simulink model "Akilli_Sayac"  (R2026b)
settings: Solver=ode23t  StopTime=t_stop  MaxStep=1e-4  RelTol=1e-4
InitFcn:
  | akilli_sayac_param
values from neighbouring files (symbols this model uses):
  bulasik_t = [0   22.5   25]    [akilli_sayac_param.m]
  bulasik_u = [0   1      0 ]    [akilli_sayac_param.m]
  camasir_t = [0   19   20.5   25]    [akilli_sayac_param.m]
  camasir_u = [0   1    0      0 ]    [akilli_sayac_param.m]
  firin_t = [0   18   19   25]    [akilli_sayac_param.m]
  firin_u = [0   1    0    0 ]    [akilli_sayac_param.m]
  k_kWh = 3600/3.6e6    (= 0.001)    [akilli_sayac_param.m]
  kap_t = [0 25]    [akilli_sayac_param.m]
  kap_u = [0 0]    [akilli_sayac_param.m]
  kettle_t = [0   7   7+10*dk   18   18+10*dk   25]    [akilli_sayac_param.m]
  kettle_u = [0   1   0         1    0          0 ]    [akilli_sayac_param.m]
  klima_t = [0   20   23   25]    [akilli_sayac_param.m]
  klima_u = [0   1    0    0 ]    [akilli_sayac_param.m]
  R_baz = Vrms^2*pf_baz^2/P_baz    (= 225.706666667)    [akilli_sayac_param.m]
  R_bulasik = Vrms^2/P_bulasik    (= 40.0757575758)    [akilli_sayac_param.m]
  R_camasir = Vrms^2*pf_camasir^2/P_camasir    (= 24.1828571429)    [akilli_sayac_param.m]
  R_firin = Vrms^2/P_firin    (= 22.0416666667)    [akilli_sayac_param.m]
  R_kettle = Vrms^2/P_kettle    (= 26.45)    [akilli_sayac_param.m]
  R_klima = Vrms^2*pf_klima^2/P_klima    (= 33.5265350877)    [akilli_sayac_param.m]
  R_tv = Vrms^2/P_tv    (= 637.34939759)    [akilli_sayac_param.m]
  T1_t = [0  6 17 25]    [akilli_sayac_param.m]
  T1_u = [0 1 0 0]    [akilli_sayac_param.m]
  T2_t = [0 17 22 25]    [akilli_sayac_param.m]
  T2_u = [0 1 0 0]    [akilli_sayac_param.m]
  T3_t = [0  6 22 25]    [akilli_sayac_param.m]
  T3_u = [1 0 1 1]    [akilli_sayac_param.m]
  t_kesme = 25    [akilli_sayac_param.m]
  tv_t = [0   19   25]    [akilli_sayac_param.m]
  tv_u = [0   1    0 ]    [akilli_sayac_param.m]
libraries: fl_lib x23, nesl_utility x11, eeRmsMeasurement x2, eePowerMeasurement x1
settings Model: Creator=Poyraz  LastModifiedBy=Poyraz
settings SimscapeCC: SimscapeLogType=all  SimscapeNominalValues="[{\"value\":\"1\",\"unit\":\"A\"},{\"value\":\"1\",\"unit\":\"bar\"},{\"value\":\"1\",\"unit\":\"cm^2\"},{\"value\":\"1\",\"unit\":\"cm^3/s\"},{\"value\":\"1\",\"unit\":\"kJ/kg\"},{\"value\":\"1\",\"unit\":\"kW\"},{\"value\":\"1\",\"unit\":\"l\"},{\"value\":\"1\",\"unit\":\"N\"},{\"value\":\"1\",\"unit\":\"N*m\"},{\"value\":\"1\",\"unit\":\"V\"},{\"value\":\"0.001\",\"unit\":\"Wb\"}]"  SimscapeUseEnergyAccounting=off

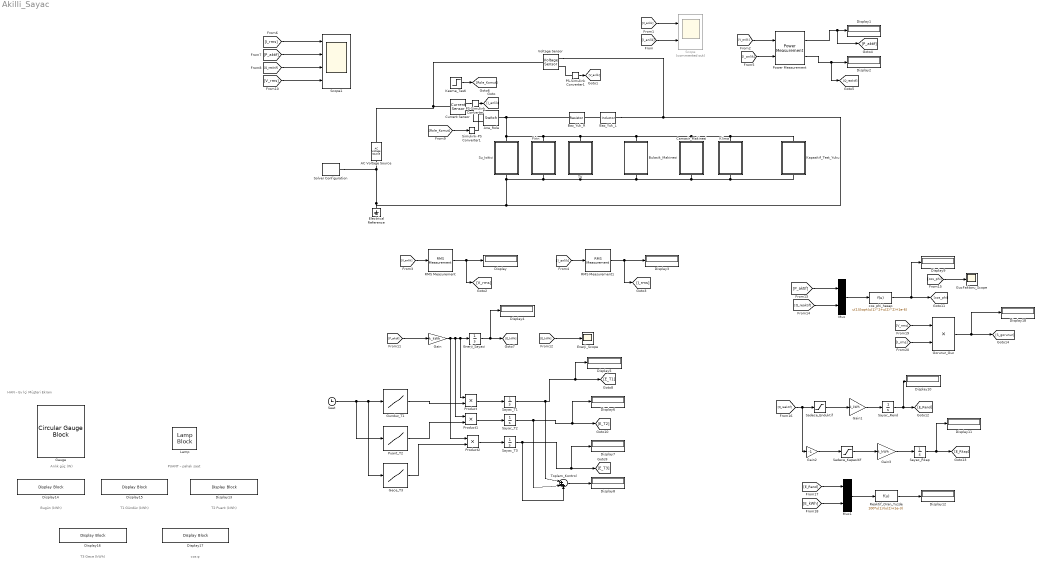
== system Akilli_Sayac ==
  note: cos φ
  note: T3 Gece (kWh)
  note: T2 Puant (kWh)
  note: T1 Gündüz (kWh)
  note: Bugün (kWh)
  note: PUANT – pahalı saat
  note: Anlık güç (W)
  note: HAN – Ev İçi Müşteri Ekranı
  AC Voltage Source : fl_lib/Electrical/Electrical Sources/AC Voltage Source  amp=Vpk V  shift=0 deg  frequency=f Hz
  Ana_Role : fl_lib/Electrical/Electrical Elements/Switch  R_closed=0.01 Ohm  G_open=1e-8 1/Ohm  Threshold=0.5  i_specify=off  i_priority=None  i=0 A  i_nominal_specify=off  i_nominal_value=1  i_nominal_unit=A  v_specify=off  v_priority=None  v=0 V  v_nominal_specify=off  v_nominal_value=1  v_nominal_unit=V
  Baz_Yuk_L : fl_lib/Electrical/Electrical Elements/Inductor  l=L_baz H  r=0 Ohm  g=1e-4 1/Ohm  i_specify=off  i_priority=None  i=0 A  i_nominal_specify=off  i_nominal_value=1  i_nominal_unit=A  v_specify=off  v_priority=None  v=0 V  v_nominal_specify=off  v_nominal_value=1  v_nominal_unit=V  i_L_specify=off  i_L_priority=High  i_L=0 A  i_L_nominal_specify=off  i_L_nominal_value=1  i_L_nominal_unit=A
  Baz_Yuk_R : fl_lib/Electrical/Electrical Elements/Resistor  R=R_baz Ohm  i_specify=off  i_priority=None  i=0 A  i_nominal_specify=off  i_nominal_value=1  i_nominal_unit=A  v_specify=off  v_priority=None  v=0 V  v_nominal_specify=off  v_nominal_value=1  v_nominal_unit=V
  Bulasik_Makinesi : Subsystem
  Camasir_Makinesi : Subsystem
  Current Sensor : fl_lib/Electrical/Electrical Sensors/Current Sensor
  Display{,1..12,18} (14 alike) : Display
  Display{13..17} (5 alike) : DisplayBlock  LabelPosition=Hide  Transparency=1  GridColor=[0.502, 0.502, 0.502]
  Electrical Reference : fl_lib/Electrical/Electrical Elements/Electrical Reference
  Enerji_Sayaci : Integrator
  Enerji_Scope : Scope
      settings: SampleTime=5e-3  ActiveDisplayYMinimum=-3.0259630448584041  ActiveDisplayYMaximum=17.0297155830163  DataLoggingVariableName=ScopeData2
  Firin : Subsystem
  Gain : Gain  Gain=k_kWh
  Gain1 : Gain  Gain=k_kWh
  Gain2 : Gain  Gain=-1
  Gain3 : Gain  Gain=k_kWh
  Gauge : CircularGaugeBlock  ScaleMax=5000  TickInterval=500  FontColor=[0.0, 0.0, 0.0]
  Gece_T3 : Lookup_n-D  NumberOfTableDimensions=1  BreakpointsForDimension1=T3_t  Table=T3_u  InterpMethod=Flat  InternalRulePriority=Speed  RndMeth=Simplest
  Gorunur_Guc : Product
  GucFaktoru_Scope : Scope
      settings: SampleTime=5e-3  ActiveDisplayYMinimum=-0.16470130830471796  ActiveDisplayYMaximum=1.1474107836524428  DataLoggingVariableName=ScopeData3
  Gunduz_T1 : Lookup_n-D  NumberOfTableDimensions=1  BreakpointsForDimension1=T1_t  Table=T1_u  InterpMethod=Flat  InternalRulePriority=Speed  RndMeth=Simplest
  Kapasitif_Test_Yuku : Subsystem
  Kesme_Testi : Step  Time=t_kesme  InitialValue=1  FinalValue=0  SampleTime=0
  Klima : Subsystem
  Lamp : LampBlock  LabelPosition=Hide  DefaultColor=[192.0, 192.0, 192.0]
  Mux : Mux  Inputs=2
  Mux1 : Mux  Inputs=2
  PS-Simulink Converter : nesl_utility/PS-Simulink Converter  PhysicalDomain=network_engine_domain  SubClassName=ps_output  LeftPortType=input  RightPortType=output  PseudoPeriodic=off  Frequencies=[]  VectorFormat=inherit  Unit=A  AffineConversion=off
  PS-Simulink Converter1 : nesl_utility/PS-Simulink Converter  PhysicalDomain=network_engine_domain  SubClassName=ps_output  LeftPortType=input  RightPortType=output  PseudoPeriodic=off  Frequencies=[]  VectorFormat=inherit  Unit=V  AffineConversion=off
  Power Measurement : eePowerMeasurement/Power Measurement  LabelModeActiveChoice=Continuous  F=f  K=[1]  Ts=0
  Product : Product
  Product1 : Product
  Product2 : Product
  Puant_T2 : Lookup_n-D  NumberOfTableDimensions=1  BreakpointsForDimension1=T2_t  Table=T2_u  InterpMethod=Flat  InternalRulePriority=Speed  RndMeth=Simplest
  RMS Measurement : eeRmsMeasurement/RMS Measurement  LabelModeActiveChoice=Total  F=f  SpecifyHarmonics=off  K=[0 1 2]  InitialRMS=0  Ts=0
      settings: LibrarySourceBlock=|
      | ee_sl_lib/Measurements/RMS
      | Measurement
  RMS Measurement1 : eeRmsMeasurement/RMS Measurement  LabelModeActiveChoice=Total  F=f  SpecifyHarmonics=off  K=[0 1 2]  InitialRMS=0  Ts=0
      settings: LibrarySourceBlock=|
      | ee_sl_lib/Measurements/RMS
      | Measurement
  Reaktif_Oran_Yuzde : Fcn  Expr=100*u(1)/(u(2)+1e-3)
  Saat : Clock
  Sadece_Enduktif : Saturate  UpperLimit=inf  LowerLimit=0
  Sadece_Kapasitif : Saturate  UpperLimit=Inf  LowerLimit=0
  Sayac_Rend : Integrator
  Sayac_Rkap : Integrator
  Sayac_T1 : Integrator
  Sayac_T2 : Integrator
  Sayac_T3 : Integrator
  Scope : Scope  Commented=on  NumInputPorts=2
      settings: ActiveDisplayYMinimum=-398.438375066242  ActiveDisplayYMaximum=373.58690131662831
  Scope1 : Scope  NumInputPorts=4
      settings: SampleTime=5e-3  ActiveDisplayYMinimum=0.41959771500038417  ActiveDisplayYMaximum=4.3103626039758209
  Simulink-PS Converter1 : nesl_utility/Simulink-PS Converter  PhysicalDomain=network_engine_domain  SubClassName=ps_input  LeftPortType=input  RightPortType=output  PseudoPeriodic=off  Frequencies=[]  NoiseDistribution=none  NoiseParameters=[]  Unit=1  AffineConversion=off  FilteringAndDerivatives=provide  SimscapeFilterOrder=1  InputFilterTimeConstant=0.001  UdotUserProvided=0
  Solver Configuration : nesl_utility/Solver Configuration  PhysicalDomain=network_engine_domain  SubClassName=solver  LeftPortType=input  RightPortType=generic  Tones=[]  Harmonics=[]  SimulateNoise=off  Profile=off  UseLocalSampling=off  EnableSwitchedLinearOptims=on  FrequencyDomain=off  UseCCode=off  RelTol=0.001  AbsTol=0.001  MinStep=1e-09  ToWorkspace=off  RevertToSquareIcSolve=off  NumHomotopyIterations=100  PhasorMode=off  PhasorModeNumHarmonics=1  ConsistencySolver=NEWTON_XTOL_AFTER_FTOL  CanonicalOrdering=CANONICAL  OptimizeIntermediates=OPTIMIZED  MulticoreSolverChoice=BACKWARD_EULER  IndexReductionMethod=DerivativeReplacement  DoDC=off  ResidualTolerance=1e-09  ConsistencyTolSource=GLOBAL  ConsistencyAbsTol=0.001  ConsistencyRelTol=0.001  ConsistencyTolFactor=0.001  UseLocalSolver=off  LocalSolverChoice=NE_BACKWARD_EULER_ADVANCER  ResolveIndetEquations=on  FunctionEvalNumThread=1  LocalSolverSampleTime=0.001  DoFixedCost=off  MaxNonlinIter=3  MaxModeIter=2  ComputeImpulses=off  ImpulseIterations=2  LinearAlgebra=auto  LinearAlgebraNumThread=0  EquationFormulation=NE_TIME_EF  DelaysMemoryBudget=1024  AutomaticFiltering=on  FilteringTimeConstant=0.001  PartitionStorageMethod=AS_NEEDED  PartitionMemoryBudget=1024  PartitionMethod=BALANCED  MultibodyUseLocalSolver=off  MultibodyLocalSolverChoice=ODE1  MultibodyLocalSolverSampleTime=0.001
  Su_Isitici : Subsystem
  TV : Subsystem
  Toplam_Kontrol : Sum  Inputs=|+++
  Voltage Sensor : fl_lib/Electrical/Electrical Sensors/Voltage Sensor
  cos_phi_hesap : Fcn  Expr=u(1)/(sqrt(u(1)^2+u(2)^2)+1e-6)
  wires:
  PS-Simulink Converter1/1 -> [V_anlik]
  PS-Simulink Converter/1 -> [I_anlik]
  [V_anlik] -> Scope/1
  [I_anlik] -> Scope/2
  [V_anlik] -> RMS Measurement/1
  [I_anlik] -> RMS Measurement1/1
  RMS Measurement/1 -> [V_rms], Display/1
  RMS Measurement1/1 -> [I_rms], Display3/1
  [I_anlik] -> Power Measurement/2
  Power Measurement/2 -> [Q_reaktif], Display2/1
  Power Measurement/1 -> [P_aktif], Display1/1
  [I_rms] -> Scope1/1
  [P_aktif] -> Scope1/2
  [Q_reaktif] -> Scope1/3
  Kesme_Testi/1 -> [Role_Komut]
  [Role_Komut] -> Simulink-PS Converter1/1
  [V_rms] -> Scope1/4
  [P_aktif] -> Gain/1
  Gain/1 -> Product2/1, Product1/1, Product/1, Enerji_Sayaci/1
  Enerji_Sayaci/1 -> Display4/1, [E_kWh]
  [E_kWh] -> Enerji_Scope/1
  [V_anlik] -> Power Measurement/1
  Saat/1 -> Puant_T2/1, Gece_T3/1, Gunduz_T1/1
  Gunduz_T1/1 -> Product/2
  Puant_T2/1 -> Product1/2
  Gece_T3/1 -> Product2/2
  Product2/1 -> Sayac_T3/1
  Product1/1 -> Sayac_T2/1
  Product/1 -> Sayac_T1/1
  Sayac_T1/1 -> Toplam_Kontrol/1, Display5/1, [E_T1]
  Sayac_T2/1 -> Toplam_Kontrol/2, Display6/1, [E_T2]
  Sayac_T3/1 -> Toplam_Kontrol/3, Display7/1, [E_T3]
  Toplam_Kontrol/1 -> Display8/1
  [P_aktif] -> Mux/1
  [Q_reaktif] -> Mux/2
  Mux/1 -> cos_phi_hesap/1
  cos_phi_hesap/1 -> Display9/1, [cos_phi]
  [cos_phi] -> GucFaktoru_Scope/1
  [Q_reaktif] -> Gain2/1, Sadece_Enduktif/1
  Sadece_Enduktif/1 -> Gain1/1
  Gain1/1 -> Sayac_Rend/1
  Sayac_Rend/1 -> Display10/1, [E_Rend]
  Gain2/1 -> Sadece_Kapasitif/1
  Sadece_Kapasitif/1 -> Gain3/1
  Gain3/1 -> Sayac_Rkap/1
  Sayac_Rkap/1 -> Display11/1, [E_Rkap]
  [E_Rend] -> Mux1/1
  [E_kWh] -> Mux1/2
  Mux1/1 -> Reaktif_Oran_Yuzde/1
  Reaktif_Oran_Yuzde/1 -> Display12/1
  [I_rms] -> Gorunur_Guc/2
  [V_rms] -> Gorunur_Guc/1
  Gorunur_Guc/1 -> Display18/1, [S_gorunur]
  connections:
  AC Voltage Source/LConn1 -- Voltage Sensor/LConn1 -- Current Sensor/LConn1
  Baz_Yuk_L/LConn1 -- Baz_Yuk_R/RConn1
  Current Sensor/RConn1 -- PS-Simulink Converter/LConn1
  PS-Simulink Converter1/LConn1 -- Voltage Sensor/RConn1
  Current Sensor/RConn2 -- Ana_Role/RConn2
  Ana_Role/LConn1 -- Kapasitif_Test_Yuku/LConn1 -- Klima/LConn1 -- Camasir_Makinesi/LConn1 -- Bulasik_Makinesi/LConn1 -- TV/LConn1 -- Firin/LConn1 -- Su_Isitici/LConn1 -- Baz_Yuk_R/LConn1
  Ana_Role/RConn1 -- Simulink-PS Converter1/RConn1
  Electrical Reference/LConn1 -- Kapasitif_Test_Yuku/RConn1 -- Klima/RConn1 -- Camasir_Makinesi/RConn1 -- Bulasik_Makinesi/RConn1 -- TV/RConn1 -- Firin/RConn1 -- Su_Isitici/RConn1 -- Baz_Yuk_L/RConn1 -- Voltage Sensor/RConn2 -- Solver Configuration/RConn1 -- AC Voltage Source/RConn1

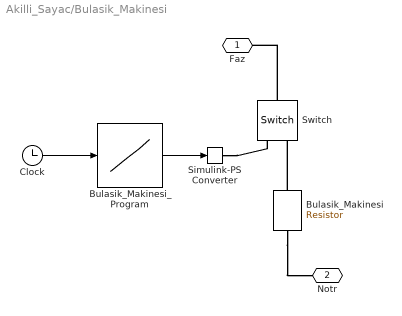
== system Akilli_Sayac/Bulasik_Makinesi ==
  Bulasik_Makinesi : fl_lib/Electrical/Electrical Elements/Resistor  R=R_bulasik Ohm  i_specify=off  i_priority=None  i=0 A  i_nominal_specify=off  i_nominal_value=1  i_nominal_unit=A  v_specify=off  v_priority=None  v=0 V  v_nominal_specify=off  v_nominal_value=1  v_nominal_unit=V
  Bulasik_Makinesi_Program : Lookup_n-D  NumberOfTableDimensions=1  BreakpointsForDimension1=bulasik_t  Table=bulasik_u  InterpMethod=Flat  InternalRulePriority=Speed  RndMeth=Simplest
  Clock : Clock
  Simulink-PS Converter : nesl_utility/Simulink-PS Converter  PhysicalDomain=network_engine_domain  SubClassName=ps_input  LeftPortType=input  RightPortType=output  PseudoPeriodic=off  Frequencies=[]  NoiseDistribution=none  NoiseParameters=[]  Unit=1  AffineConversion=off  FilteringAndDerivatives=provide  SimscapeFilterOrder=1  InputFilterTimeConstant=0.001  UdotUserProvided=0
  Switch : fl_lib/Electrical/Electrical Elements/Switch  R_closed=0.01 Ohm  G_open=1e-8 1/Ohm  Threshold=0.5  i_specify=off  i_priority=None  i=0 A  i_nominal_specify=off  i_nominal_value=1  i_nominal_unit=A  v_specify=off  v_priority=None  v=0 V  v_nominal_specify=off  v_nominal_value=1  v_nominal_unit=V
  Faz : PMIOPort  Side=Left
  Notr : PMIOPort  Port=2  Side=Right
  wires:
  Clock/1 -> Bulasik_Makinesi_Program/1
  Bulasik_Makinesi_Program/1 -> Simulink-PS Converter/1
  connections:
  Bulasik_Makinesi/RConn1 -- Notr/RConn1
  Bulasik_Makinesi/LConn1 -- Switch/RConn2
  Switch/LConn1 -- Faz/RConn1
  Simulink-PS Converter/RConn1 -- Switch/RConn1

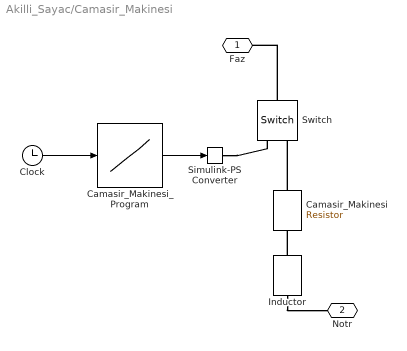
== system Akilli_Sayac/Camasir_Makinesi ==
  Camasir_Makinesi : fl_lib/Electrical/Electrical Elements/Resistor  R=R_camasir Ohm  i_specify=off  i_priority=None  i=0 A  i_nominal_specify=off  i_nominal_value=1  i_nominal_unit=A  v_specify=off  v_priority=None  v=0 V  v_nominal_specify=off  v_nominal_value=1  v_nominal_unit=V
  Camasir_Makinesi_Program : Lookup_n-D  NumberOfTableDimensions=1  BreakpointsForDimension1=camasir_t  Table=camasir_u  InterpMethod=Flat  InternalRulePriority=Speed  RndMeth=Simplest
  Clock : Clock
  Inductor : fl_lib/Electrical/Electrical Elements/Inductor  l=L_camasir H  r=0 Ohm  g=1e-4 1/Ohm  i_specify=off  i_priority=None  i=0 A  i_nominal_specify=off  i_nominal_value=1  i_nominal_unit=A  v_specify=off  v_priority=None  v=0 V  v_nominal_specify=off  v_nominal_value=1  v_nominal_unit=V  i_L_specify=off  i_L_priority=High  i_L=0 A  i_L_nominal_specify=off  i_L_nominal_value=1  i_L_nominal_unit=A
  Simulink-PS Converter : nesl_utility/Simulink-PS Converter  PhysicalDomain=network_engine_domain  SubClassName=ps_input  LeftPortType=input  RightPortType=output  PseudoPeriodic=off  Frequencies=[]  NoiseDistribution=none  NoiseParameters=[]  Unit=1  AffineConversion=off  FilteringAndDerivatives=provide  SimscapeFilterOrder=1  InputFilterTimeConstant=0.001  UdotUserProvided=0
  Switch : fl_lib/Electrical/Electrical Elements/Switch  R_closed=0.01 Ohm  G_open=1e-8 1/Ohm  Threshold=0.5  i_specify=off  i_priority=None  i=0 A  i_nominal_specify=off  i_nominal_value=1  i_nominal_unit=A  v_specify=off  v_priority=None  v=0 V  v_nominal_specify=off  v_nominal_value=1  v_nominal_unit=V
  Faz : PMIOPort  Side=Left
  Notr : PMIOPort  Port=2  Side=Right
  wires:
  Clock/1 -> Camasir_Makinesi_Program/1
  Camasir_Makinesi_Program/1 -> Simulink-PS Converter/1
  connections:
  Camasir_Makinesi/LConn1 -- Switch/RConn2
  Switch/LConn1 -- Faz/RConn1
  Simulink-PS Converter/RConn1 -- Switch/RConn1
  Inductor/LConn1 -- Camasir_Makinesi/RConn1
  Inductor/RConn1 -- Notr/RConn1

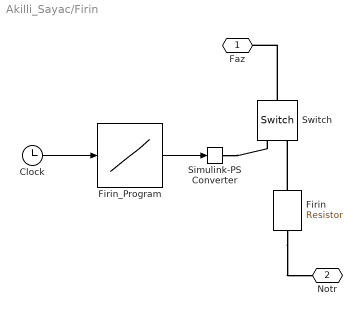
== system Akilli_Sayac/Firin ==
  Clock : Clock
  Firin : fl_lib/Electrical/Electrical Elements/Resistor  R=R_firin Ohm  i_specify=off  i_priority=None  i=0 A  i_nominal_specify=off  i_nominal_value=1  i_nominal_unit=A  v_specify=off  v_priority=None  v=0 V  v_nominal_specify=off  v_nominal_value=1  v_nominal_unit=V
  Firin_Program : Lookup_n-D  NumberOfTableDimensions=1  BreakpointsForDimension1=firin_t  Table=firin_u  InterpMethod=Flat  InternalRulePriority=Speed  RndMeth=Simplest
  Simulink-PS Converter : nesl_utility/Simulink-PS Converter  PhysicalDomain=network_engine_domain  SubClassName=ps_input  LeftPortType=input  RightPortType=output  PseudoPeriodic=off  Frequencies=[]  NoiseDistribution=none  NoiseParameters=[]  Unit=1  AffineConversion=off  FilteringAndDerivatives=provide  SimscapeFilterOrder=1  InputFilterTimeConstant=0.001  UdotUserProvided=0
  Switch : fl_lib/Electrical/Electrical Elements/Switch  R_closed=0.01 Ohm  G_open=1e-8 1/Ohm  Threshold=0.5  i_specify=off  i_priority=None  i=0 A  i_nominal_specify=off  i_nominal_value=1  i_nominal_unit=A  v_specify=off  v_priority=None  v=0 V  v_nominal_specify=off  v_nominal_value=1  v_nominal_unit=V
  Faz : PMIOPort  Side=Left
  Notr : PMIOPort  Port=2  Side=Right
  wires:
  Clock/1 -> Firin_Program/1
  Firin_Program/1 -> Simulink-PS Converter/1
  connections:
  Firin/RConn1 -- Notr/RConn1
  Firin/LConn1 -- Switch/RConn2
  Switch/LConn1 -- Faz/RConn1
  Simulink-PS Converter/RConn1 -- Switch/RConn1

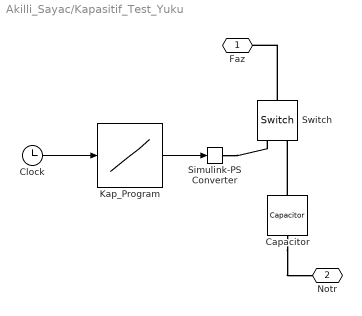
== system Akilli_Sayac/Kapasitif_Test_Yuku ==
  Capacitor : fl_lib/Electrical/Electrical Elements/Capacitor  c=C_kap F  r=1e-6 Ohm  g=0 1/Ohm  i_specify=off  i_priority=None  i=0 A  i_nominal_specify=off  i_nominal_value=1  i_nominal_unit=A  v_specify=off  v_priority=None  v=0 V  v_nominal_specify=off  v_nominal_value=1  v_nominal_unit=V  vc_specify=off  vc_priority=High  vc=0 V  vc_nominal_specify=off  vc_nominal_value=1  vc_nominal_unit=V
  Clock : Clock
  Kap_Program : Lookup_n-D  NumberOfTableDimensions=1  BreakpointsForDimension1=kap_t  Table=kap_u  InterpMethod=Flat  InternalRulePriority=Speed  RndMeth=Simplest
  Simulink-PS Converter : nesl_utility/Simulink-PS Converter  PhysicalDomain=network_engine_domain  SubClassName=ps_input  LeftPortType=input  RightPortType=output  PseudoPeriodic=off  Frequencies=[]  NoiseDistribution=none  NoiseParameters=[]  Unit=1  AffineConversion=off  FilteringAndDerivatives=provide  SimscapeFilterOrder=1  InputFilterTimeConstant=0.001  UdotUserProvided=0
  Switch : fl_lib/Electrical/Electrical Elements/Switch  R_closed=0.01 Ohm  G_open=1e-8 1/Ohm  Threshold=0.5  i_specify=off  i_priority=None  i=0 A  i_nominal_specify=off  i_nominal_value=1  i_nominal_unit=A  v_specify=off  v_priority=None  v=0 V  v_nominal_specify=off  v_nominal_value=1  v_nominal_unit=V
  Faz : PMIOPort  Side=Left
  Notr : PMIOPort  Port=2  Side=Right
  wires:
  Clock/1 -> Kap_Program/1
  Kap_Program/1 -> Simulink-PS Converter/1
  connections:
  Switch/LConn1 -- Faz/RConn1
  Simulink-PS Converter/RConn1 -- Switch/RConn1
  Capacitor/LConn1 -- Switch/RConn2
  Capacitor/RConn1 -- Notr/RConn1

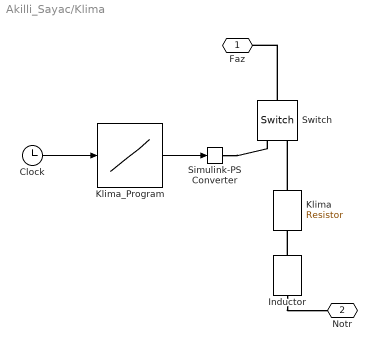
== system Akilli_Sayac/Klima ==
  Clock : Clock
  Inductor : fl_lib/Electrical/Electrical Elements/Inductor  l=L_klima H  r=0 Ohm  g=1e-4 1/Ohm  i_specify=off  i_priority=None  i=0 A  i_nominal_specify=off  i_nominal_value=1  i_nominal_unit=A  v_specify=off  v_priority=None  v=0 V  v_nominal_specify=off  v_nominal_value=1  v_nominal_unit=V  i_L_specify=off  i_L_priority=High  i_L=0 A  i_L_nominal_specify=off  i_L_nominal_value=1  i_L_nominal_unit=A
  Klima : fl_lib/Electrical/Electrical Elements/Resistor  R=R_klima Ohm  i_specify=off  i_priority=None  i=0 A  i_nominal_specify=off  i_nominal_value=1  i_nominal_unit=A  v_specify=off  v_priority=None  v=0 V  v_nominal_specify=off  v_nominal_value=1  v_nominal_unit=V
  Klima_Program : Lookup_n-D  NumberOfTableDimensions=1  BreakpointsForDimension1=klima_t  Table=klima_u  InterpMethod=Flat  InternalRulePriority=Speed  RndMeth=Simplest
  Simulink-PS Converter : nesl_utility/Simulink-PS Converter  PhysicalDomain=network_engine_domain  SubClassName=ps_input  LeftPortType=input  RightPortType=output  PseudoPeriodic=off  Frequencies=[]  NoiseDistribution=none  NoiseParameters=[]  Unit=1  AffineConversion=off  FilteringAndDerivatives=provide  SimscapeFilterOrder=1  InputFilterTimeConstant=0.001  UdotUserProvided=0
  Switch : fl_lib/Electrical/Electrical Elements/Switch  R_closed=0.01 Ohm  G_open=1e-8 1/Ohm  Threshold=0.5  i_specify=off  i_priority=None  i=0 A  i_nominal_specify=off  i_nominal_value=1  i_nominal_unit=A  v_specify=off  v_priority=None  v=0 V  v_nominal_specify=off  v_nominal_value=1  v_nominal_unit=V
  Faz : PMIOPort  Side=Left
  Notr : PMIOPort  Port=2  Side=Right
  wires:
  Clock/1 -> Klima_Program/1
  Klima_Program/1 -> Simulink-PS Converter/1
  connections:
  Klima/LConn1 -- Switch/RConn2
  Switch/LConn1 -- Faz/RConn1
  Simulink-PS Converter/RConn1 -- Switch/RConn1
  Inductor/LConn1 -- Klima/RConn1
  Inductor/RConn1 -- Notr/RConn1

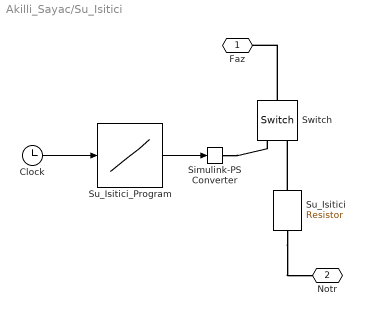
== system Akilli_Sayac/Su_Isitici ==
  Clock : Clock
  Simulink-PS Converter : nesl_utility/Simulink-PS Converter  PhysicalDomain=network_engine_domain  SubClassName=ps_input  LeftPortType=input  RightPortType=output  PseudoPeriodic=off  Frequencies=[]  NoiseDistribution=none  NoiseParameters=[]  Unit=1  AffineConversion=off  FilteringAndDerivatives=provide  SimscapeFilterOrder=1  InputFilterTimeConstant=0.001  UdotUserProvided=0
  Su_Isitici : fl_lib/Electrical/Electrical Elements/Resistor  R=R_kettle Ohm  i_specify=off  i_priority=None  i=0 A  i_nominal_specify=off  i_nominal_value=1  i_nominal_unit=A  v_specify=off  v_priority=None  v=0 V  v_nominal_specify=off  v_nominal_value=1  v_nominal_unit=V
  Su_Isitici_Program : Lookup_n-D  NumberOfTableDimensions=1  BreakpointsForDimension1=kettle_t  Table=kettle_u  InterpMethod=Flat  InternalRulePriority=Speed  RndMeth=Simplest
  Switch : fl_lib/Electrical/Electrical Elements/Switch  R_closed=0.01 Ohm  G_open=1e-8 1/Ohm  Threshold=0.5  i_specify=off  i_priority=None  i=0 A  i_nominal_specify=off  i_nominal_value=1  i_nominal_unit=A  v_specify=off  v_priority=None  v=0 V  v_nominal_specify=off  v_nominal_value=1  v_nominal_unit=V
  Faz : PMIOPort  Side=Left
  Notr : PMIOPort  Port=2  Side=Right
  wires:
  Clock/1 -> Su_Isitici_Program/1
  Su_Isitici_Program/1 -> Simulink-PS Converter/1
  connections:
  Su_Isitici/RConn1 -- Notr/RConn1
  Su_Isitici/LConn1 -- Switch/RConn2
  Switch/LConn1 -- Faz/RConn1
  Simulink-PS Converter/RConn1 -- Switch/RConn1

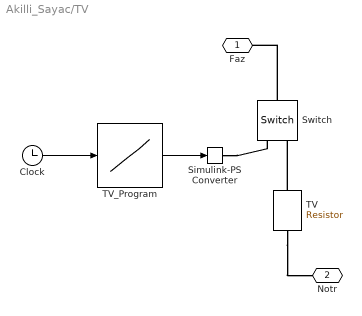
== system Akilli_Sayac/TV ==
  Clock : Clock
  Simulink-PS Converter : nesl_utility/Simulink-PS Converter  PhysicalDomain=network_engine_domain  SubClassName=ps_input  LeftPortType=input  RightPortType=output  PseudoPeriodic=off  Frequencies=[]  NoiseDistribution=none  NoiseParameters=[]  Unit=1  AffineConversion=off  FilteringAndDerivatives=provide  SimscapeFilterOrder=1  InputFilterTimeConstant=0.001  UdotUserProvided=0
  Switch : fl_lib/Electrical/Electrical Elements/Switch  R_closed=0.01 Ohm  G_open=1e-8 1/Ohm  Threshold=0.5  i_specify=off  i_priority=None  i=0 A  i_nominal_specify=off  i_nominal_value=1  i_nominal_unit=A  v_specify=off  v_priority=None  v=0 V  v_nominal_specify=off  v_nominal_value=1  v_nominal_unit=V
  TV : fl_lib/Electrical/Electrical Elements/Resistor  R=R_tv Ohm  i_specify=off  i_priority=None  i=0 A  i_nominal_specify=off  i_nominal_value=1  i_nominal_unit=A  v_specify=off  v_priority=None  v=0 V  v_nominal_specify=off  v_nominal_value=1  v_nominal_unit=V
  TV_Program : Lookup_n-D  NumberOfTableDimensions=1  BreakpointsForDimension1=tv_t  Table=tv_u  InterpMethod=Flat  InternalRulePriority=Speed  RndMeth=Simplest
  Faz : PMIOPort  Side=Left
  Notr : PMIOPort  Port=2  Side=Right
  wires:
  Clock/1 -> TV_Program/1
  TV_Program/1 -> Simulink-PS Converter/1
  connections:
  TV/RConn1 -- Notr/RConn1
  TV/LConn1 -- Switch/RConn2
  Switch/LConn1 -- Faz/RConn1
  Simulink-PS Converter/RConn1 -- Switch/RConn1
